simulink model "squawk4_openloop"  (R2025a)
settings: Solver=ode45  StartTime=0.0  StopTime=600  MaxStep=0.05  RelTol=1e-6  AbsTol=1e-8
values from neighbouring files (symbols this model uses):
  Keng = diag([1, r2d/u0, r2d, r2d])    [squawk4_lab.m]
  x0 = [10; 0; 0; 0]    [squawk4_lab.m]
undefined symbols (not defined in the file or in its folder): A, B, C, D
settings Model: Creator=rtydf  LastModifiedBy=rtydf

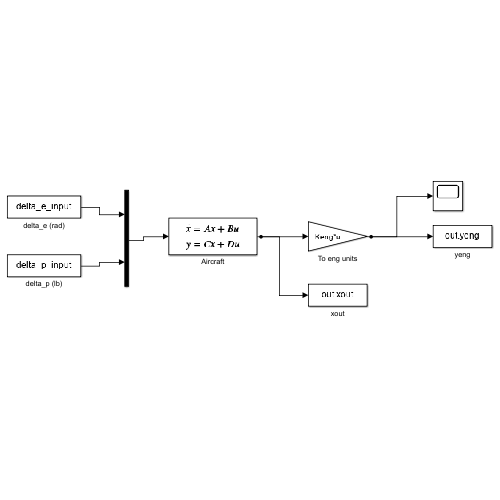
[thumbnail: Simulink's stored preview of the top-level diagram]
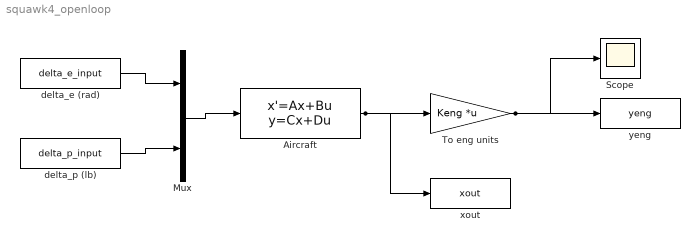
== system squawk4_openloop ==
  Aircraft : StateSpace  A=A  B=B  C=C  D=D  InitialCondition=x0
  Mux : Mux  Inputs=2
  Scope : Scope
  To eng units : Gain  Gain=Keng  Multiplication=Matrix(K*u)
  delta_e (rad) : FromWorkspace  VariableName=delta_e_input
  delta_p (lb) : FromWorkspace  VariableName=delta_p_input
  xout : ToWorkspace  VariableName=xout  SaveFormat=Timeseries  SampleTime=-1
  yeng : ToWorkspace  VariableName=yeng  SaveFormat=Timeseries  SampleTime=-1
  wires:
  delta_e (rad)/1 -> Mux/1
  delta_p (lb)/1 -> Mux/2
  Mux/1 -> Aircraft/1
  Aircraft/1 -> To eng units/1, xout/1
  To eng units/1 -> Scope/1, yeng/1
